simulink model "ConfiguredHevMmVirtualVehicle"  (R2025b)
settings: configuration reference "VehicleVariable" (kept outside this file)
StartFcn:
  | %tic
StopFcn:
  | %toc
model workspace (MAT data in the model file):
  ExtDrvCmdsSwitch : Simulink.Parameter (value not decoded)
  ExtDrvRefSwitch : Simulink.Parameter (value not decoded)
  ExtEnvSwitch : Simulink.Parameter (value not decoded)
  ExtGndSwitch : Simulink.Parameter (value not decoded)
symbols that are objects in the model workspace (value not decoded): ExtDrvCmdsSwitch, ExtDrvRefSwitch, ExtEnvSwitch, ExtGndSwitch
undefined symbols (not defined in the file or in its folder): AmbTemp, BaroPress, CurvGradRef, CurvRef, DCM, DriverAeroRes, DriverDrivelineRes, DriverInitialGear, DriverPreviewDist, DriverRollRes, DriverShiftTime, DriverTimeConst, DriverTractiveForce, EnvAbsPrs, EnvAirTemp, EnvGrvty, EnvNomFrictionScaling, EnvNominalGrade, EnvScnFrictionMap, EnvScnFrictionMapXBpts, EnvScnFrictionMapYBpts, EnvScnHeightMap, EnvScnHeightMapXBpts, EnvScnHeightMapYBpts, EnvWindVelX, EnvWindVelY, EnvWindVelZ, Gnd, Grade, HazzardCmd, HighBeamCmd, lambda_mux, LeftSignalCmd, LngRef, LowBeamCmd, LtrRef, PhiRef, PlntVehDstCGFrntAxl, PlntVehDstCGRearAxl, PlntVehInitLatPos, PlntVehInitLongPos, PlntVehInitPitchAng, PlntVehInitRollAng, PlntVehInitVertPos, PlntVehInitYawAng, PlntVehMass, PlntVehTrckWdth, PlntVehYawMomentInertia, PlntWhlLdRadiusFrnt, PlntWhlLdRadiusRear, RightSignalCmd, ScnCRRadius, Sim3dSensor, Wind, XRef, YRef, Z
libraries: simulink x28, autolibutils x8, autolibsharedcommon x7, vehdynlibscenariocommon x7, vehdynlibviscommon x4, vehdynlibdriver x2, sim3dgroundtruthsensorlib x2, sim3dlib x2, autolibshared x2, sim3dautolib x2, sl3dlib x1, sharedtransform x1
(part 2 of 6)

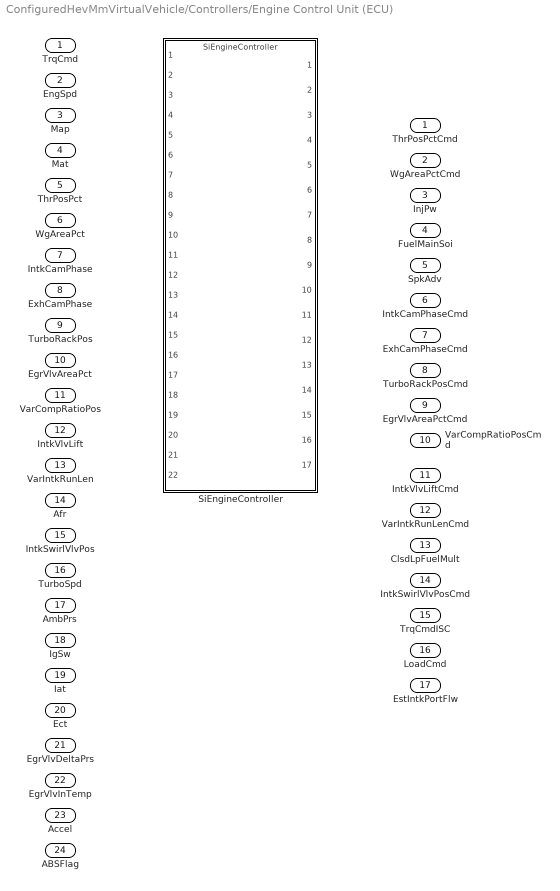
== system ConfiguredHevMmVirtualVehicle/Controllers/Engine Control Unit (ECU) ==
  TrqCmd : Inport
  EngSpd : Inport  Port=2
  Map : Inport  Port=3
  Mat : Inport  Port=4
  ThrPosPct : Inport  Port=5
  WgAreaPct : Inport  Port=6
  IntkCamPhase : Inport  Port=7
  ExhCamPhase : Inport  Port=8
  TurboRackPos : Inport  Port=9
  EgrVlvAreaPct : Inport  Port=10
  VarCompRatioPos : Inport  Port=11
  IntkVlvLift : Inport  Port=12
  VarIntkRunLen : Inport  Port=13
  Afr : Inport  Port=14
  IntkSwirlVlvPos : Inport  Port=15
  TurboSpd : Inport  Port=16  Unit=rpm
  AmbPrs : Inport  Port=17
  IgSw : Inport  Port=18
  Iat : Inport  Port=19
  Ect : Inport  Port=20
  EgrVlvDeltaPrs : Inport  Port=21
  EgrVlvInTemp : Inport  Port=22
  Accel : Inport  Port=23
  ABSFlag : Inport  Port=24
  SiEngineController : ModelReference  ModelNameDialog=SiEngineController  SimulationMode=Normal  VariantControl=SiEngineController  ModelReferenceVersion=11.0
  ThrPosPctCmd : Outport  VectorParamsAs1DForOutWhenUnconnected=off
  WgAreaPctCmd : Outport  Port=2  VectorParamsAs1DForOutWhenUnconnected=off
  InjPw : Outport  Port=3  VectorParamsAs1DForOutWhenUnconnected=off
  FuelMainSoi : Outport  Port=4  VectorParamsAs1DForOutWhenUnconnected=off
  SpkAdv : Outport  Port=5  VectorParamsAs1DForOutWhenUnconnected=off
  IntkCamPhaseCmd : Outport  Port=6  VectorParamsAs1DForOutWhenUnconnected=off
  ExhCamPhaseCmd : Outport  Port=7  VectorParamsAs1DForOutWhenUnconnected=off
  TurboRackPosCmd : Outport  Port=8  VectorParamsAs1DForOutWhenUnconnected=off
  EgrVlvAreaPctCmd : Outport  Port=9  VectorParamsAs1DForOutWhenUnconnected=off
  VarCompRatioPosCmd : Outport  Port=10  VectorParamsAs1DForOutWhenUnconnected=off
  IntkVlvLiftCmd : Outport  Port=11  VectorParamsAs1DForOutWhenUnconnected=off
  VarIntkRunLenCmd : Outport  Port=12  VectorParamsAs1DForOutWhenUnconnected=off
  ClsdLpFuelMult : Outport  Port=13  VectorParamsAs1DForOutWhenUnconnected=off
  IntkSwirlVlvPosCmd : Outport  Port=14  VectorParamsAs1DForOutWhenUnconnected=off
  TrqCmdISC : Outport  Port=15  VectorParamsAs1DForOutWhenUnconnected=off
  LoadCmd : Outport  Port=16  VectorParamsAs1DForOutWhenUnconnected=off
  EstIntkPortFlw : Outport  Port=17  VectorParamsAs1DForOutWhenUnconnected=off

== system ConfiguredHevMmVirtualVehicle/Controllers/TCU Input ==
  CntrlRx : Inport
  Brake : Inport  Port=2
  Bus Selector : BusSelector  OutputSignals=ABSFlag
  Bus Selector1 : BusSelector  OutputSignals=Driver.AccelFdbk,Driver.DecelFdbk,Driver.GearFdbk,Trans.Info.Eng.EngSpd,FrntWheels.Wheels.Omega,RearWheels.Wheels.Omega,Body.BdyFrm.Cg.Vel.xdot
  Bus to Vector : BusToVector
  Bus to Vector1 : BusToVector
  Ground : Ground
  Ground1 : Ground
  Rate Transition{1..8,23} (9 alike) : RateTransition  Deterministic=off
  Vector Concatenate : Concatenate
  <AccFdbk> : Outport
  <DecelFdbk> : Outport  Port=2
  <GearFdbk> : Outport  Port=3
  <EngSpd> : Outport  Port=4
  <Omega> : Outport  Port=5
  <Vehicle> : Outport  Port=6
  ABSFlag : Outport  Port=7
  UpReq : Outport  Port=8
  DnReq : Outport  Port=9
  wires:
  Bus Selector1/7 -> Rate Transition5/1  "<xdot>"
  Bus Selector1/2 -> Rate Transition1/1  "<DecelFdbk>"
  Ground/1 -> Rate Transition7/1
  CntrlRx/1 -> Bus Selector1/1
  Bus Selector1/1 -> Rate Transition23/1  "<AccelFdbk>"
  Vector Concatenate/1 -> Rate Transition4/1
  Bus Selector1/4 -> Rate Transition3/1  "<EngSpd>"
  Bus Selector1/3 -> Rate Transition2/1  "<GearFdbk>"
  Ground1/1 -> Rate Transition8/1
  Bus Selector/1 -> Rate Transition6/1  "<ABSFlag>"
  Brake/1 -> Bus Selector/1
  Rate Transition23/1 -> <AccFdbk>/1
  Rate Transition1/1 -> <DecelFdbk>/1
  Rate Transition2/1 -> <GearFdbk>/1
  Rate Transition3/1 -> <EngSpd>/1
  Rate Transition4/1 -> <Omega>/1
  Rate Transition5/1 -> <Vehicle>/1
  Rate Transition6/1 -> ABSFlag/1
  Rate Transition7/1 -> UpReq/1
  Rate Transition8/1 -> DnReq/1
  Bus Selector1/5 -> Bus to Vector/1  "<Omega>"
  Bus Selector1/6 -> Bus to Vector1/1  "<Omega>"
  Bus to Vector/1 -> Vector Concatenate/1
  Bus to Vector1/1 -> Vector Concatenate/2

== system ConfiguredHevMmVirtualVehicle/Controllers/TCU Output ==
  GearCmd : Inport
  Bus Creator1 : BusCreator  Inputs=1
  First Order Hold : FirstOrderHold  ErrorTolerance=inf
  Trans : Outport
  wires:
  Bus Creator1/1 -> Trans/1  "Trans"
  GearCmd/1 -> First Order Hold/1  "GearCmd"
  First Order Hold/1 -> Bus Creator1/1  "GearCmd"

== system ConfiguredHevMmVirtualVehicle/Controllers/Thermal Input ==
  Bus Element In : Inport  PortName=CntrlRx  Element=Thermal.BattCoolTemp
  Bus Element In2 : Inport  PortName=CntrlRx  Element=Thermal.CondPress
  Bus Element In5 : Inport  PortName=CntrlRx  Element=Thermal.MotorTemp
  Bus Element In6 : Inport  PortName=CntrlRx  Element=Thermal.BattTemp
  Bus Element In7 : Inport  PortName=CntrlRx  Element=Thermal.EMCoolTempOut
  BusElementIn2 : Inport  PortName=CntrlRx  Element=Thermal.ChlrPress
  Bus Element In1 : Inport  PortName=CntrlRx  Element=Battery.BMSSensors.CellTemperatures
  Bus Element In4 : Inport  PortName=CntrlRx  Element=Env.AmbTemp
  Rate Transition{,1,3..6,8,11} (8 alike) : RateTransition
  CoolTemp : Outport
  CellTemps : Outport  Port=2
  AmbTemp : Outport  Port=3
  CondPress : Outport  Port=4
  MotorTemp : Outport  Port=5
  BattTemp : Outport  Port=6
  EMCoolTempOut : Outport  Port=7
  ChlrPress : Outport  Port=8
  wires:
  Bus Element In/1 -> Rate Transition/1
  Bus Element In1/1 -> Rate Transition8/1
  Rate Transition/1 -> CoolTemp/1
  Bus Element In2/1 -> Rate Transition1/1
  Rate Transition1/1 -> CondPress/1
  Rate Transition3/1 -> AmbTemp/1
  Bus Element In4/1 -> Rate Transition3/1
  Rate Transition4/1 -> MotorTemp/1
  Bus Element In5/1 -> Rate Transition4/1
  Rate Transition5/1 -> BattTemp/1
  Bus Element In6/1 -> Rate Transition5/1
  Rate Transition6/1 -> EMCoolTempOut/1
  Bus Element In7/1 -> Rate Transition6/1
  Rate Transition8/1 -> CellTemps/1
  BusElementIn2/1 -> Rate Transition11/1
  Rate Transition11/1 -> ChlrPress/1

== system ConfiguredHevMmVirtualVehicle/Controllers/Thermal Management ==
  CoolTemp : Inport
  CellTemps : Inport  Port=2
  AmbTemp : Inport  Port=3  Unit=K
  CondPress : Inport  Port=4
  MotorTemp : Inport  Port=5
  BattTemp : Inport  Port=6
  EMCoolTempOut : Inport  Port=7
  ChlrPress : Inport  Port=8
  NoThermalControl : ModelReference  ModelNameDialog=NoThermalControl  SimulationMode=Normal  VariantControl=NoThermalControl  ModelReferenceVersion=5.0
  ValveCmd : Outport
  PumpCmd : Outport  Port=2
  CmpCmd : Outport  Port=3
  FanCmd : Outport  Port=4
  HeaterCmd : Outport  Port=5
  MotPmpCmd : Outport  Port=6
  BattPmpCmd : Outport  Port=7
  ChlrByPCmd : Outport  Port=8
  SerParCmd : Outport  Port=9
  RadByPCmd : Outport  Port=10

== system ConfiguredHevMmVirtualVehicle/Controllers/Thermal Output ==
  ValveCmd : Inport
  PumpCmd : Inport  Port=2
  CmpCmd : Inport  Port=3
  FanCmd : Inport  Port=4
  HeaterCmd : Inport  Port=5
  MotPmpCmd : Inport  Port=6
  BattPmpCmd : Inport  Port=7
  ChlrPyPCmd : Inport  Port=8
  SerParCmd : Inport  Port=9
  RadByPCmd : Inport  Port=10
  First Order Hold{,1..9} (10 alike) : FirstOrderHold  ErrorTolerance=inf
  Bus Element Out : Outport  PortName=Thermal  Element=ValveCmd
  Bus Element Out1 : Outport  PortName=Thermal  Element=PumpCmd
  Bus Element Out2 : Outport  PortName=Thermal  Element=CmpCmd
  Bus Element Out3 : Outport  PortName=Thermal  Element=FanCmd
  Bus Element Out4 : Outport  PortName=Thermal  Element=HeaterCmd
  Bus Element Out5 : Outport  PortName=Thermal  Element=MotPmpCmd
  Bus Element Out6 : Outport  PortName=Thermal  Element=BattPmpCmd
  Bus Element Out7 : Outport  PortName=Thermal  Element=ChlrByPCmd
  Bus Element Out8 : Outport  PortName=Thermal  Element=SerParCmd
  Bus Element Out9 : Outport  PortName=Thermal  Element=RadByPCmd
  wires:
  PumpCmd/1 -> First Order Hold1/1
  ValveCmd/1 -> First Order Hold/1
  First Order Hold/1 -> Bus Element Out/1
  First Order Hold1/1 -> Bus Element Out1/1
  CmpCmd/1 -> First Order Hold2/1
  First Order Hold2/1 -> Bus Element Out2/1
  First Order Hold3/1 -> Bus Element Out3/1
  FanCmd/1 -> First Order Hold3/1
  HeaterCmd/1 -> First Order Hold4/1
  First Order Hold4/1 -> Bus Element Out4/1
  MotPmpCmd/1 -> First Order Hold5/1
  First Order Hold5/1 -> Bus Element Out5/1
  BattPmpCmd/1 -> First Order Hold6/1
  First Order Hold6/1 -> Bus Element Out6/1
  ChlrPyPCmd/1 -> First Order Hold7/1
  First Order Hold7/1 -> Bus Element Out7/1
  First Order Hold8/1 -> Bus Element Out8/1
  SerParCmd/1 -> First Order Hold8/1
  First Order Hold9/1 -> Bus Element Out9/1
  RadByPCmd/1 -> First Order Hold9/1

== system ConfiguredHevMmVirtualVehicle/Controllers/Transmission Control Unit (TCU) ==
  Accel : Inport
  BrkCmd : Inport  Port=2
  GearReq : Inport  Port=3
  EngSpd : Inport  Port=4
  Omega : Inport  Port=5  Unit=rad/s
  VehSpdFdbk : Inport  Port=6
  ABSFlag : Inport  Port=7
  UpReq : Inport  Port=8
  DownReq : Inport  Port=9  Unit=rad/s
  DriverPassThrough : ModelReference  ModelNameDialog=DriverPassThrough  SimulationMode=Normal  VariantControl=DriverPassThrough  ModelReferenceVersion=11.0
  " Gear" : Outport  VectorParamsAs1DForOutWhenUnconnected=off

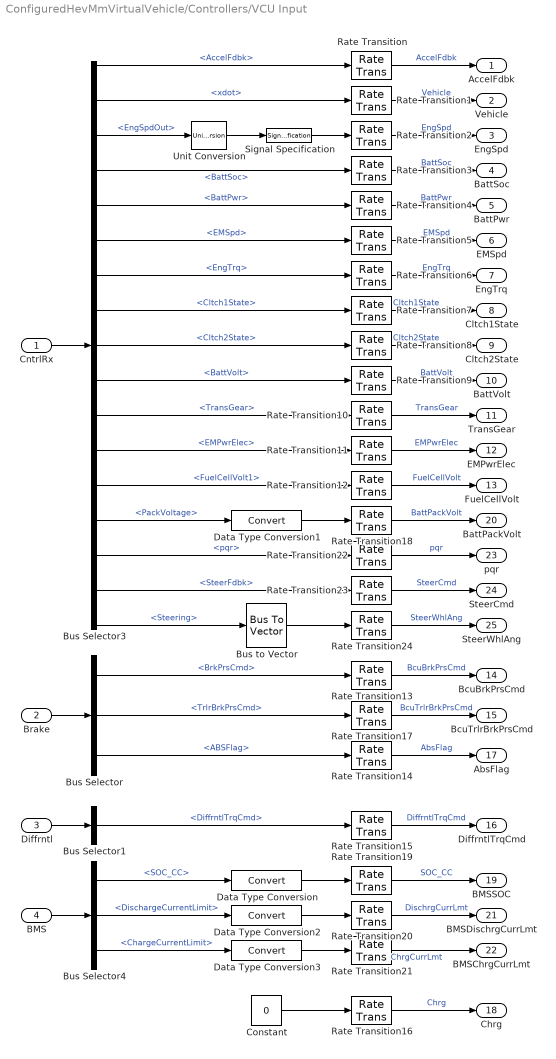
== system ConfiguredHevMmVirtualVehicle/Controllers/VCU Input ==
  CntrlRx : Inport
  Brake : Inport  Port=2
  Diffrntl : Inport  Port=3
  BMS : Inport  Port=4
  Bus Selector : BusSelector  OutputSignals=BrkPrsCmd,TrlrBrkPrsCmd,ABSFlag
  Bus Selector1 : BusSelector  OutputSignals=DiffrntlTrqCmd
  Bus Selector3 : BusSelector  OutputSignals=Driver.AccelFdbk,Body.BdyFrm.Cg.Vel.xdot,Engine.EngSpdOut,Battery.BattInfo.BattSoc,Battery.BattInfo.BattPwr,EM.EMSpd,Engine.EngTrq,Trans.Cltch1State,Trans.Cltch2State,Battery.BattInfo.BattVolt,Trans.Info.Trans.TransGear,EM.EMPwrElec,FuelCell.FuelCellVolt1,Battery.BMSSensors.PackVoltage,IMU.pqr,Driver.SteerFdbk,Steering
  Bus Selector4 : BusSelector  OutputSignals=BMSInfo.SOC.SOC_CC,BMSCmd.CurrentLimitsBus.DischargeCurrentLimit,BMSCmd.CurrentLimitsBus.ChargeCurrentLimit
  Bus to Vector : BusToVector
  Constant : Constant  Value=0  SampleTime=-1
  Data Type Conversion{,1..3} (4 alike) : DataTypeConversion  SaturateOnIntegerOverflow=off  RndMeth=Floor
  Rate Transition{,1..24} (25 alike) : RateTransition  Deterministic=off
  Signal Specification : SignalSpecification  Unit=rad/s
  Unit Conversion : UnitConversion
  AccelFdbk : Outport
  Vehicle : Outport  Port=2
  EngSpd : Outport  Port=3
  BattSoc : Outport  Port=4
  BattPwr : Outport  Port=5
  EMSpd : Outport  Port=6
  EngTrq : Outport  Port=7
  Cltch1State : Outport  Port=8
  Cltch2State : Outport  Port=9
  BattVolt : Outport  Port=10
  TransGear : Outport  Port=11
  EMPwrElec : Outport  Port=12
  FuelCellVolt : Outport  Port=13
  BcuBrkPrsCmd : Outport  Port=14
  BcuTrlrBrkPrsCmd : Outport  Port=15
  DiffrntlTrqCmd : Outport  Port=16
  AbsFlag : Outport  Port=17
  Chrg : Outport  Port=18
  BMSSOC : Outport  Port=19
  BattPackVolt : Outport  Port=20
  BMSDischrgCurrLmt : Outport  Port=21
  BMSChrgCurrLmt : Outport  Port=22
  pqr : Outport  Port=23
  SteerCmd : Outport  Port=24
  SteerWhlAng : Outport  Port=25
  wires:
  Bus Selector3/5 -> Rate Transition4/1  "<BattPwr>"
  Bus Selector3/1 -> Rate Transition/1  "<AccelFdbk>"
  Bus Selector3/7 -> Rate Transition6/1  "<EngTrq>"
  Bus Selector3/4 -> Rate Transition3/1  "<BattSoc>"
  Bus Selector3/6 -> Rate Transition5/1  "<EMSpd>"
  CntrlRx/1 -> Bus Selector3/1
  Bus Selector3/11 -> Rate Transition10/1  "<TransGear>"
  Bus Selector3/9 -> Rate Transition8/1  "<Cltch2State>"
  Bus Selector3/13 -> Rate Transition12/1  "<FuelCellVolt1>"
  Bus Selector3/2 -> Rate Transition1/1  "<xdot>"
  Bus Selector3/8 -> Rate Transition7/1  "<Cltch1State>"
  Bus Selector3/10 -> Rate Transition9/1  "<BattVolt>"
  Bus Selector3/3 -> Unit Conversion/1  "<EngSpdOut>"
  Bus Selector3/12 -> Rate Transition11/1  "<EMPwrElec>"
  Bus Selector/1 -> Rate Transition13/1  "<BrkPrsCmd>"
  Constant/1 -> Rate Transition16/1
  Brake/1 -> Bus Selector/1
  Bus Selector/3 -> Rate Transition14/1  "<ABSFlag>"
  Diffrntl/1 -> Bus Selector1/1
  Bus Selector1/1 -> Rate Transition15/1  "<DiffrntlTrqCmd>"
  Rate Transition/1 -> AccelFdbk/1  "AccelFdbk"
  Rate Transition1/1 -> Vehicle/1  "Vehicle"
  Rate Transition2/1 -> EngSpd/1  "EngSpd"
  Rate Transition3/1 -> BattSoc/1  "BattSoc"
  Rate Transition4/1 -> BattPwr/1  "BattPwr"
  Rate Transition5/1 -> EMSpd/1  "EMSpd"
  Rate Transition6/1 -> EngTrq/1  "EngTrq"
  Rate Transition7/1 -> Cltch1State/1  "Cltch1State"
  Rate Transition8/1 -> Cltch2State/1  "Cltch2State"
  Rate Transition9/1 -> BattVolt/1  "BattVolt"
  Rate Transition10/1 -> TransGear/1  "TransGear"
  Rate Transition11/1 -> EMPwrElec/1  "EMPwrElec"
  Rate Transition12/1 -> FuelCellVolt/1  "FuelCellVolt"
  Rate Transition13/1 -> BcuBrkPrsCmd/1  "BcuBrkPrsCmd"
  Rate Transition14/1 -> AbsFlag/1  "AbsFlag"
  Rate Transition15/1 -> DiffrntlTrqCmd/1  "DiffrntlTrqCmd"
  Rate Transition16/1 -> Chrg/1  "Chrg"
  Rate Transition20/1 -> BMSDischrgCurrLmt/1  "DischrgCurrLmt"
  Rate Transition19/1 -> BMSSOC/1  "SOC_CC"
  Rate Transition21/1 -> BMSChrgCurrLmt/1  "ChrgCurrLmt"
  Data Type Conversion3/1 -> Rate Transition21/1
  Data Type Conversion2/1 -> Rate Transition20/1
  Bus Selector4/1 -> Data Type Conversion/1  "<SOC_CC>"
  Data Type Conversion/1 -> Rate Transition19/1
  Bus Selector4/3 -> Data Type Conversion3/1  "<ChargeCurrentLimit>"
  Bus Selector4/2 -> Data Type Conversion2/1  "<DischargeCurrentLimit>"
  BMS/1 -> Bus Selector4/1
  Data Type Conversion1/1 -> Rate Transition18/1
  Rate Transition18/1 -> BattPackVolt/1  "BattPackVolt"
  Bus Selector3/14 -> Data Type Conversion1/1  "<PackVoltage>"
  Bus Selector/2 -> Rate Transition17/1  "<TrlrBrkPrsCmd>"
  Rate Transition17/1 -> BcuTrlrBrkPrsCmd/1  "BcuTrlrBrkPrsCmd"
  Rate Transition22/1 -> pqr/1  "pqr"
  Rate Transition23/1 -> SteerCmd/1  "SteerCmd"
  Rate Transition24/1 -> SteerWhlAng/1  "SteerWhlAng"
  Bus Selector3/15 -> Rate Transition22/1  "<pqr>"
  Bus Selector3/16 -> Rate Transition23/1  "<SteerFdbk>"
  Bus Selector3/17 -> Bus to Vector/1  "<Steering>"
  Unit Conversion/1 -> Signal Specification/1
  Signal Specification/1 -> Rate Transition2/1
  Bus to Vector/1 -> Rate Transition24/1

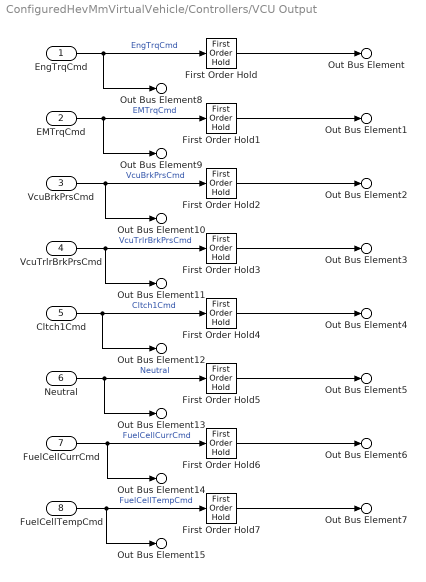
== system ConfiguredHevMmVirtualVehicle/Controllers/VCU Output ==
  EngTrqCmd : Inport
  EMTrqCmd : Inport  Port=2
  VcuBrkPrsCmd : Inport  Port=3
  VcuTrlrBrkPrsCmd : Inport  Port=4
  Cltch1Cmd : Inport  Port=5
  Neutral : Inport  Port=6
  FuelCellCurrCmd : Inport  Port=7
  FuelCellTempCmd : Inport  Port=8
  First Order Hold{,1..2,4..7} (7 alike) : FirstOrderHold  ErrorTolerance=inf
  First Order Hold3 : FirstOrderHold  ErrorTolerance=inf  AllowContinuousInput=on
  Out Bus Element : Outport  PortName=Vcu  Element=EngTrqCmd
  Out Bus Element1 : Outport  PortName=Vcu  Element=EMTrqCmd
  Out Bus Element2 : Outport  PortName=Vcu  Element=VcuBrkPrsCmd
  Out Bus Element3 : Outport  PortName=Vcu  Element=VcuTrlrBrkPrsCmd
  Out Bus Element4 : Outport  PortName=Vcu  Element=Cltch1Cmd
  Out Bus Element5 : Outport  PortName=Vcu  Element=Neutral
  Out Bus Element6 : Outport  PortName=Vcu  Element=FuelCellCurrCmd
  Out Bus Element7 : Outport  PortName=Vcu  Element=FuelCellTempCmd
  Out Bus Element8 : Outport  Port=2  PortName=VcuFdbk  Element=EngTrqCmd
  Out Bus Element9 : Outport  Port=2  PortName=VcuFdbk  Element=EMTrqCmd
  Out Bus Element10 : Outport  Port=2  PortName=VcuFdbk  Element=VcuBrkPrsCmd
  Out Bus Element11 : Outport  Port=2  PortName=VcuFdbk  Element=VcuTrlrBrkPrsCmd
  Out Bus Element12 : Outport  Port=2  PortName=VcuFdbk  Element=Cltch1Cmd
  Out Bus Element13 : Outport  Port=2  PortName=VcuFdbk  Element=Neutral
  Out Bus Element14 : Outport  Port=2  PortName=VcuFdbk  Element=FuelCellCurrCmd
  Out Bus Element15 : Outport  Port=2  PortName=VcuFdbk  Element=FuelCellTempCmd
  wires:
  Cltch1Cmd/1 -> Out Bus Element12/1, First Order Hold4/1  "Cltch1Cmd"
  EngTrqCmd/1 -> Out Bus Element8/1, First Order Hold/1  "EngTrqCmd"
  VcuBrkPrsCmd/1 -> Out Bus Element10/1, First Order Hold2/1  "VcuBrkPrsCmd"
  Neutral/1 -> Out Bus Element13/1, First Order Hold5/1  "Neutral"
  FuelCellCurrCmd/1 -> Out Bus Element14/1, First Order Hold6/1  "FuelCellCurrCmd"
  EMTrqCmd/1 -> Out Bus Element9/1, First Order Hold1/1  "EMTrqCmd"
  FuelCellTempCmd/1 -> Out Bus Element15/1, First Order Hold7/1  "FuelCellTempCmd"
  VcuTrlrBrkPrsCmd/1 -> Out Bus Element11/1, First Order Hold3/1  "VcuTrlrBrkPrsCmd"
  First Order Hold/1 -> Out Bus Element/1
  First Order Hold1/1 -> Out Bus Element1/1
  First Order Hold2/1 -> Out Bus Element2/1
  First Order Hold3/1 -> Out Bus Element3/1
  First Order Hold4/1 -> Out Bus Element4/1
  First Order Hold5/1 -> Out Bus Element5/1
  First Order Hold6/1 -> Out Bus Element6/1
  First Order Hold7/1 -> Out Bus Element7/1

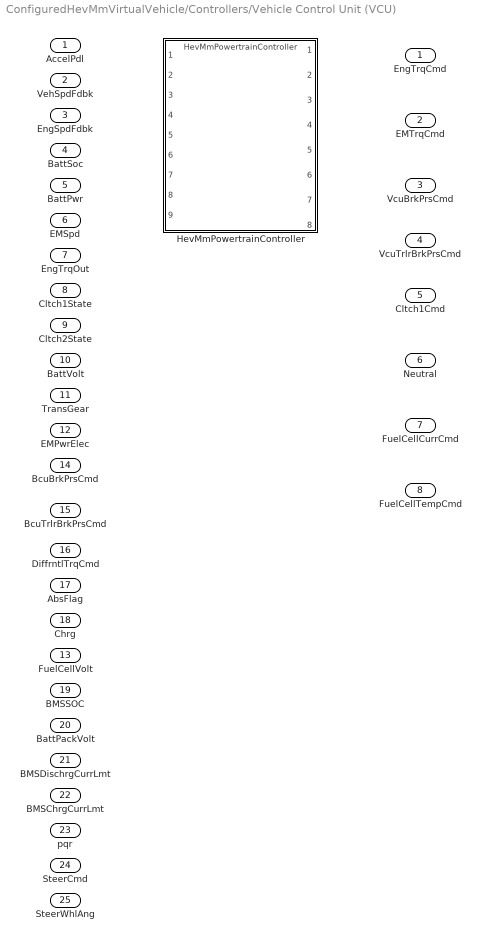
== system ConfiguredHevMmVirtualVehicle/Controllers/Vehicle Control Unit (VCU) ==
  AccelPdl : Inport
  VehSpdFdbk : Inport  Port=2
  EngSpdFdbk : Inport  Port=3
  BattSoc : Inport  Port=4
  BattPwr : Inport  Port=5
  EMSpd : Inport  Port=6
  EngTrqOut : Inport  Port=7
  Cltch1State : Inport  Port=8
  Cltch2State : Inport  Port=9
  BattVolt : Inport  Port=10
  TransGear : Inport  Port=11
  EMPwrElec : Inport  Port=12
  FuelCellVolt : Inport  Port=13
  BcuBrkPrsCmd : Inport  Port=14
  BcuTrlrBrkPrsCmd : Inport  Port=15
  DiffrntlTrqCmd : Inport  Port=16
  AbsFlag : Inport  Port=17
  Chrg : Inport  Port=18
  BMSSOC : Inport  Port=19
  BattPackVolt : Inport  Port=20
  BMSDischrgCurrLmt : Inport  Port=21
  BMSChrgCurrLmt : Inport  Port=22
  pqr : Inport  Port=23
  SteerCmd : Inport  Port=24
  SteerWhlAng : Inport  Port=25
  HevMmPowertrainController : ModelReference  ModelNameDialog=HevMmPowertrainController  SimulationMode=Normal  VariantControl=HevMmPowertrainController  ModelReferenceVersion=16.0
  EngTrqCmd : Outport  VectorParamsAs1DForOutWhenUnconnected=off
  EMTrqCmd : Outport  Port=2  VectorParamsAs1DForOutWhenUnconnected=off
  VcuBrkPrsCmd : Outport  Port=3  VectorParamsAs1DForOutWhenUnconnected=off
  VcuTrlrBrkPrsCmd : Outport  Port=4  VectorParamsAs1DForOutWhenUnconnected=off
  Cltch1Cmd : Outport  Port=5  VectorParamsAs1DForOutWhenUnconnected=off
  Neutral : Outport  Port=6  VectorParamsAs1DForOutWhenUnconnected=off
  FuelCellCurrCmd : Outport  Port=7  VectorParamsAs1DForOutWhenUnconnected=off
  FuelCellTempCmd : Outport  Port=8  VectorParamsAs1DForOutWhenUnconnected=off

== system ConfiguredHevMmVirtualVehicle/Driver Commands/Driver Commands ==
  VehRef : Inport
  VehFdbk : Inport  Port=2
  Env : Inport  Port=3
  SteerCmd : Inport  Port=4
  AccelCmd : Inport  Port=5
  BrakeCmd : Inport  Port=6
  GearCmd : Inport  Port=7
  Dashboard Widgets : Subsystem  VariantControl=Dashboard Widgets
  Game Wheel Hardware : Subsystem  VariantControl=Game Wheel Hardware
  Longitudinal Driver : Subsystem  VariantControl=Longitudinal Driver
  No Driver : Subsystem  VariantControl=No Driver
  Open Loop : Subsystem  VariantControl=Open Loop
  Predictive Driver : Subsystem  VariantControl=Predictive Driver
  Predictive Stanley Driver : Subsystem  VariantControl=Predictive Stanley Driver
  " Driver" : Outport  VectorParamsAs1DForOutWhenUnconnected=off

== system ConfiguredHevMmVirtualVehicle/Environment/Ground Feedback ==
  WheelFdbk : Inport
  InertFrm : Inport  Port=2
  3D Engine : Subsystem  VariantControl=1
  Constant : Subsystem  VariantControl=0
  Height Map : Subsystem  VariantControl=3
  Ideal Inclined Plane : Subsystem  VariantControl=4
  Three-Axle Constant : Subsystem  VariantControl=2
  Z : Outport  VectorParamsAs1DForOutWhenUnconnected=off
  DCM : Outport  Port=2  VectorParamsAs1DForOutWhenUnconnected=off

== system ConfiguredHevMmVirtualVehicle/Environment/Subsystem ==
  ExtEnv : Inport
  ExtGnd : Inport  Port=2
  AmbTemp : Inport  Port=3
  BaroPress : Inport  Port=4
  Wind : Inport  Port=5
  InGnd : Inport  Port=6
  Bus Assignment : BusAssignment  AssignedSignals=AmbTemp,BaroPress,Wind,Grade
  Bus Assignment1 : BusAssignment  AssignedSignals=Z,DCM,lambda_mux
  Bus Assignment2 : BusAssignment  AssignedSignals=BaroPress,AmbTemp,Wind,Grade,Gnd
  Bus Selector : BusSelector  OutputSignals=BaroPress,AmbTemp,Wind,Grade
  Estimated Grade : Subsystem
  ExtEnvSwitch : Constant  Value=ExtEnvSwitch  SampleTime=-1
  ExtGndSwitch : Constant  Value=ExtGndSwitch  SampleTime=-1
  Switch : Switch  Criteria=u2 > Threshold  SaturateOnIntegerOverflow=off  InputSameDT=off
  Switch1 : Switch  Criteria=u2 > Threshold  SaturateOnIntegerOverflow=off  InputSameDT=off
  To Virtual Bus : SignalConversion  ConversionOutput=Virtual bus  OverrideOpt=off
  VVCEnv : Constant  Value=0  OutDataTypeStr=Bus: VVCEnvGndBUS  SampleTime=-1
  Variant Subsystem : Subsystem  Variant=on  VariantControlMode=label  LabelModeActiveChoice=TwoAxle
  Env : Outport
  wires:
  Bus Assignment1/1 -> Switch1/3
  Estimated Grade/1(Grade) -> Bus Assignment/5
  ExtGndSwitch/1 -> Switch1/2
  ExtEnv/1 -> Switch/1, Bus Assignment/1
  InGnd/1 -> Variant Subsystem/1(InGnd), Estimated Grade/1(Gnd)
  ExtEnvSwitch/1 -> Switch/2
  Bus Assignment/1 -> Switch/3
  BaroPress/1 -> Bus Assignment/3
  VVCEnv/1 -> Bus Assignment2/1
  Switch1/1 -> Bus Assignment2/6
  ExtGnd/1 -> Switch1/1, Bus Assignment1/1
  Wind/1 -> Bus Assignment/4
  Bus Selector/1 -> Bus Assignment2/2  "<BaroPress>"
  Switch/1 -> Bus Selector/1
  Bus Selector/2 -> Bus Assignment2/3  "<AmbTemp>"
  Bus Assignment2/1 -> To Virtual Bus/1
  Bus Selector/4 -> Bus Assignment2/5  "<Grade>"
  Bus Selector/3 -> Bus Assignment2/4  "<Wind>"
  AmbTemp/1 -> Bus Assignment/2
  To Virtual Bus/1 -> Env/1
  Variant Subsystem/1(z) -> Bus Assignment1/2
  Variant Subsystem/2(<DCM>) -> Bus Assignment1/3
  Variant Subsystem/3(lambda_mux) -> Bus Assignment1/4

== system ConfiguredHevMmVirtualVehicle/Environment/Varying Friction ==
  InertFrm : Inport
  Cg : Inport  Port=2
  Constant Friction : Subsystem  VariantControl=0
  Friction Map : Subsystem  VariantControl=3
  Three-Axle Constant Friction : Subsystem  VariantControl=2
  Varying Friction : Subsystem  VariantControl=1
  FricCoeffLambda : Outport

== system ConfiguredHevMmVirtualVehicle/Scenarios/Coordinate Systems ==
  ExtDrvRefIn : Inport
  ExtDrvCmdIn : Inport  Port=2
  ISO 8855 (Z-up) : Subsystem  VariantControl=Choice
  SAE J670 (Z-down) : Subsystem  VariantControl=ISO 8855 (Z-up)1
  ExtDrvRef : Outport
  ExtDrvCmd : Outport  Port=2

== system ConfiguredHevMmVirtualVehicle/Scenarios/Reference Generator ==
  note: 1) Add Subsystem or Model blocks as valid variant choices.
      | 2) You cannot connect blocks at this level. At simulation, connectivity is automatically
      | determined, based on the active variant and port name matching.
  "VehFdbk " : Inport
  Braking : Subsystem  VariantControl=Braking
  Constant Radius : Subsystem  VariantControl=Constant Radius
  Double Lane Change : Subsystem  VariantControl=Double Lane Change
  Drive Cycle : Subsystem  VariantControl=Drive Cycle
  Fishhook : Subsystem  VariantControl=Fishhook
  Increasing Steer : Subsystem  VariantControl=Increasing Steer
  No Commands : Subsystem  VariantControl=No Commands
  Sine with Dwell : Subsystem  VariantControl=Sine with Dwell
  Swept Sine : Subsystem  VariantControl=Swept Sine
  WOT : Subsystem  VariantControl=Wide Open Throttle
  DrvRef : Outport  VectorParamsAs1DForOutWhenUnconnected=off
  DrvCmd : Outport  Port=2  VectorParamsAs1DForOutWhenUnconnected=off
  " Vis" : Outport  Port=3  VectorParamsAs1DForOutWhenUnconnected=off
  " Fdbk" : Outport  Port=4  VectorParamsAs1DForOutWhenUnconnected=off

== system ConfiguredHevMmVirtualVehicle/Scenarios/Reference Routing ==
  ExtDrvRef : Inport  OutDataTypeStr=Bus: VVCDrvRefBUS
  ExtDrvCmds : Inport  Port=2  OutDataTypeStr=Bus: VVCDrvCmdBUS
  DrvRef : Inport  Port=3
  DrvCmd : Inport  Port=4
  Bus Assignment : BusAssignment  AssignedSignals=LngRef,LtrRef,XRef,YRef,PhiRef,CurvRef
  Bus Assignment1 : BusAssignment  AssignedSignals=SteerCmd.EnblSteerCmd,SteerCmd.SteerCmd,SteerCmd.SteerHld,SteerCmd.SteerZero,AccelCmd.EnblAccelCmd,AccelCmd.AccelCmd,AccelCmd.AccelHld,AccelCmd.AccelZero,DecelCmd.EnblDecelCmd,DecelCmd.DecelCmd,DecelCmd.DecelHld,DecelCmd.DecelZero,TransCmd.TransModeCmd,TransCmd.GearCmd,TransCmd.UpShiftCmd,TransCmd.DwnShiftCmd,TransCmd.ClutchCmd
  Bus Creator : BusCreator  Inputs=2
  Bus Selector : BusSelector  OutputSignals=LngRef,LtrRef,XRef,YRef,PhiRef,CurvRef
  Bus Selector1 : BusSelector  OutputSignals=SteerCmd.EnblSteerCmd,SteerCmd.SteerCmd,SteerCmd.SteerHld,SteerCmd.SteerZero,AccelCmd.EnableAccelCmd,AccelCmd.AccelCmd,AccelCmd.AccelHld,AccelCmd.AccelZero,DecelCmd.EnblDecelCmd,DecelCmd.DecelCmd,DecelCmd.DecelHld,DecelCmd.DecelZero,TransCmd.TransModeCmd,TransCmd.GearCmd,TransCmd.UpShiftCmd,TransCmd.DwnShiftCmd,TransCmd.ClutchCmd
  ExtDrvCmdsSwitch : Constant  Value=ExtDrvCmdsSwitch
  ExtDrvRefSwitch : Constant  Value=ExtDrvRefSwitch
  Switch : Switch  Criteria=u2 > Threshold  SaturateOnIntegerOverflow=off  InputSameDT=off
  Switch1 : Switch  Criteria=u2 > Threshold  SaturateOnIntegerOverflow=off  InputSameDT=off
  Unit Conversion1 : UnitConversion
  VehRef : Outport
  wires:
  Bus Selector1/9 -> Bus Assignment1/10  "<EnblDecelCmd>"
  Bus Selector/1 -> Bus Assignment/2  "<LngRef>"
  Bus Selector1/8 -> Bus Assignment1/9  "<AccelZero>"
  Bus Selector1/4 -> Bus Assignment1/5  "<SteerZero>"
  Bus Selector1/3 -> Bus Assignment1/4  "<SteerHld>"
  Bus Selector1/10 -> Bus Assignment1/11  "<DecelCmd>"
  ExtDrvRef/1 -> Bus Assignment/1, Switch/1
  Bus Selector1/1 -> Bus Assignment1/2  "<EnblSteerCmd>"
  Bus Assignment/1 -> Switch/3
  Bus Assignment1/1 -> Switch1/3
  Bus Selector/2 -> Bus Assignment/3  "<LtrRef>"
  Bus Selector1/7 -> Bus Assignment1/8  "<AccelHld>"
  DrvRef/1 -> Bus Selector/1
  Switch1/1 -> Bus Creator/2  "DrvCmd"
  Bus Selector1/12 -> Bus Assignment1/13  "<DecelZero>"
  Bus Selector1/11 -> Bus Assignment1/12  "<DecelHld>"
  Bus Selector1/2 -> Unit Conversion1/1  "<SteerCmd>"
  Bus Selector1/6 -> Bus Assignment1/7  "<AccelCmd>"
  ExtDrvCmds/1 -> Bus Assignment1/1, Switch1/1
  ExtDrvRefSwitch/1 -> Switch/2
  ExtDrvCmdsSwitch/1 -> Switch1/2
  Switch/1 -> Bus Creator/1  "DrvRef"
  Bus Selector/6 -> Bus Assignment/7  "<CurvRef>"
  Bus Selector1/5 -> Bus Assignment1/6  "<EnableAccelCmd>"
  Bus Creator/1 -> VehRef/1  "VehRef"
  Unit Conversion1/1 -> Bus Assignment1/3
  DrvCmd/1 -> Bus Selector1/1
  Bus Selector/3 -> Bus Assignment/4  "<XRef>"
  Bus Selector/4 -> Bus Assignment/5  "<YRef>"
  Bus Selector/5 -> Bus Assignment/6  "<PhiRef>"
  Bus Selector1/13 -> Bus Assignment1/14  "<TransModeCmd>"
  Bus Selector1/14 -> Bus Assignment1/15  "<GearCmd>"
  Bus Selector1/15 -> Bus Assignment1/16  "<UpShiftCmd>"
  Bus Selector1/16 -> Bus Assignment1/17  "<DwnShiftCmd>"
  Bus Selector1/17 -> Bus Assignment1/18  "<ClutchCmd>"

== system ConfiguredHevMmVirtualVehicle/Visualization/3D Engine ==
  note: 1) Add Subsystem or Model blocks as valid variant choices.
      | 2) You cannot connect blocks at this level. At simulation, connectivity is automatically
      | determined, based on the active variant and port name matching.
  VehFdbk : Inport
  3D Engine : Subsystem  VariantControl=Engine3D
  3D Engine Disabled : Subsystem  VariantControl=NoEngine3D

== system ConfiguredHevMmVirtualVehicle/Visualization/Coordinate Systems ==
  VehFdbkIn : Inport
  ISO 8855 (Z-up) : Subsystem  VariantControl=Choice
  SAE J670 (Z-down) : Subsystem  VariantControl=ISO 8855 (Z-up)1
  VehFdbk : Outport

== system ConfiguredHevMmVirtualVehicle/Visualization/DataLogging ==
  VehFdbk : Inport
  Bus Selector : BusSelector  OutputSignals=Battery.BattInfo.BattSoc,Battery.BattInfo.BattVolt,Battery.BattInfo.BattCurr,Body.BdyFrm.Cg.Vel.xdot,Body.BdyFrm.Cg.Acc.ax,Body.BdyFrm.Cg.Acc.ay,Body.BdyFrm.Cg.Acc.az,Driver.SteerFdbk,Driver.AccelFdbk,Driver.DecelFdbk,Driver.GearFdbk,EM.EMSpd,EM.EMTrq,Engine.EngTrq,Engine.EngSpdOut
  Terminator{,1..14} (15 alike) : Terminator
  wires:
  Bus Selector/2 -> Terminator1/1  "<BattVolt>"
  VehFdbk/1 -> Bus Selector/1
  Bus Selector/1 -> Terminator/1  "<BattSoc>"
  Bus Selector/4 -> Terminator3/1  "<xdot>"
  Bus Selector/6 -> Terminator5/1  "<ay>"
  Bus Selector/9 -> Terminator8/1  "<AccelFdbk>"
  Bus Selector/5 -> Terminator4/1  "<ax>"
  Bus Selector/3 -> Terminator2/1  "<BattCurr>"
  Bus Selector/15 -> Terminator14/1  "<EngSpdOut>"
  Bus Selector/11 -> Terminator10/1  "<GearFdbk>"
  Bus Selector/7 -> Terminator6/1  "<az>"
  Bus Selector/12 -> Terminator11/1  "<EMSpd>"
  Bus Selector/8 -> Terminator7/1  "<SteerFdbk>"
  Bus Selector/14 -> Terminator13/1  "<EngTrq>"
  Bus Selector/10 -> Terminator9/1  "<DecelFdbk>"
  Bus Selector/13 -> Terminator12/1  "<EMTrq>"

== system ConfiguredHevMmVirtualVehicle/Visualization/Emission Calculations ==
  VehSpd : Inport
  TP HC Mass Flow : Inport  Port=2
  TP CO Mass Flow : Inport  Port=3
  TP NOx Mass Flow : Inport  Port=4
  TP CO2 Mass Flow : Inport  Port=5
  Integrator{,1..4} (5 alike) : Integrator
  Kg to g : Gain  Gain=1000
  "Kg to g " : Gain  Gain=1000
  "Kg to g  " : Gain  Gain=1000
  "Kg to g   " : Gain  Gain=1000
  L/100 Km Calc{,1..3} (4 alike) : Product  Inputs=/*
  Rate Transition{,1..3} (4 alike) : RateTransition  Deterministic=off
  Saturation : Saturate  UpperLimit=Inf  LowerLimit=0.2  ZeroCross=off
  Saturation1 : Saturate  UpperLimit=Inf  LowerLimit=1  ZeroCross=off
  Signal Specification5 : SignalSpecification  Unit=m/s
  Unit Conversion5 : UnitConversion
  m to km : Gain  Gain=0.001
  m to mi : Gain  Gain=0.000621371
  TP HC Mass : Outport  VectorParamsAs1DForOutWhenUnconnected=off
  TP CO Mass : Outport  Port=2  VectorParamsAs1DForOutWhenUnconnected=off
  TP NOx Mass : Outport  Port=3  VectorParamsAs1DForOutWhenUnconnected=off
  TP CO2 Mass : Outport  Port=4  VectorParamsAs1DForOutWhenUnconnected=off
  wires:
  L/100 Km Calc/1 -> Rate Transition/1
  m to mi/1 -> Saturation/1
  Saturation/1 -> L/100 Km Calc2/1, L/100 Km Calc1/1, L/100 Km Calc/1
  TP HC Mass Flow/1 -> Integrator1/1
  Integrator1/1 -> Kg to g/1
  Integrator/1 -> m to km/1, m to mi/1
  Kg to g/1 -> L/100 Km Calc/2
  TP CO Mass Flow/1 -> Integrator2/1
  Integrator2/1 -> "Kg to g "/1
  "Kg to g "/1 -> L/100 Km Calc1/2
  TP NOx Mass Flow/1 -> Integrator3/1
  Integrator3/1 -> "Kg to g  "/1
  "Kg to g  "/1 -> L/100 Km Calc2/2
  L/100 Km Calc1/1 -> Rate Transition1/1
  L/100 Km Calc2/1 -> Rate Transition2/1
  TP CO2 Mass Flow/1 -> Integrator4/1
  Integrator4/1 -> "Kg to g   "/1
  "Kg to g   "/1 -> L/100 Km Calc3/2
  L/100 Km Calc3/1 -> Rate Transition3/1
  Saturation1/1 -> L/100 Km Calc3/1
  m to km/1 -> Saturation1/1
  Rate Transition/1 -> TP HC Mass/1  "TP HC Mass (g/mi)"
  Rate Transition1/1 -> TP CO Mass/1  "TP CO Mass (g/mi)"
  Rate Transition2/1 -> TP NOx Mass/1  "TP NOx Mass (g/mi)"
  Rate Transition3/1 -> TP CO2 Mass/1  "TP CO2 Mass (g/km)"
  Unit Conversion5/1 -> Signal Specification5/1
  VehSpd/1 -> Unit Conversion5/1
  Signal Specification5/1 -> Integrator/1

== system ConfiguredHevMmVirtualVehicle/Visualization/External Output Routing ==
  VehFdbk : Inport
  Bus Assignment : BusAssignment  AssignedSignals=Driver.SteerFdbk,Driver.AccelFdbk,Driver.DecelFdbk,Driver.GearFdbk,Driver.IgnFdbk,Driveline.EngSpd,Driveline.TransGear,Body.InertFrm.Cg.Disp.X,Body.InertFrm.Cg.Disp.Y,Body.InertFrm.Cg.Disp.Z,Body.InertFrm.Cg.Vel.Xdot,Body.InertFrm.Cg.Vel.Ydot,Body.InertFrm.Cg.Vel.Zdot,Body.InertFrm.Cg.Ang.phi,Body.InertFrm.Cg.Ang.theta,Body.InertFrm.Cg.Ang.psi,Body.InertFrm.Geom.Disp.X,Body.InertFrm.Geom.Disp.Y,Body.InertFrm.Geom.Disp.Z,Body.InertFrm.Geom.Vel.Xdot,Body.InertFrm.Geom.Vel.Ydot,Body.InertFrm.Geom.Vel.Zdot,Body.BdyFrm.Cg.Vel.xdot,Body.BdyFrm.Cg.Vel.ydot,Body.BdyFrm.Cg.Vel.zdot,Body.BdyFrm.Cg.AngVel.p,Body.BdyFrm.Cg.AngVel.q,Body.BdyFrm.Cg.AngVel.r,Body.BdyFrm.Cg.Acc.ax,Body.BdyFrm.Cg.Acc.ay,Body.BdyFrm.Cg.Acc.az,Body.BdyFrm.Cg.Acc.xddot,Body.BdyFrm.Cg.Acc.yddot,Body.BdyFrm.Cg.Acc.zddot,Body.BdyFrm.Cg.AngAcc.pdot,Body.BdyFrm.Cg.AngAcc.qdot,Body.BdyFrm.Cg.AngAcc.rdot
  Bus Selector1 : BusSelector  OutputSignals=Driver.SteerFdbk,Driver.AccelFdbk,Driver.DecelFdbk,Driver.GearFdbk,Driver.IgnFdbk
  Bus Selector2 : BusSelector  OutputSignals=Body.InertFrm.Cg.Disp.X,Body.InertFrm.Cg.Disp.Y,Body.InertFrm.Cg.Disp.Z,Body.InertFrm.Cg.Vel.Xdot,Body.InertFrm.Cg.Vel.Ydot,Body.InertFrm.Cg.Vel.Zdot,Body.InertFrm.Cg.Ang.phi,Body.InertFrm.Cg.Ang.theta,Body.InertFrm.Cg.Ang.psi,Body.InertFrm.Geom.Disp.X,Body.InertFrm.Geom.Disp.Y,Body.InertFrm.Geom.Disp.Z,Body.InertFrm.Geom.Vel.Xdot,Body.InertFrm.Geom.Vel.Ydot,Body.InertFrm.Geom.Vel.Zdot,Body.BdyFrm.Cg.Vel.xdot,Body.BdyFrm.Cg.Vel.ydot,Body.BdyFrm.Cg.Vel.zdot,Body.BdyFrm.Cg.AngVel.p,Body.BdyFrm.Cg.AngVel.q,Body.BdyFrm.Cg.AngVel.r,Body.BdyFrm.Cg.Acc.ax,Body.BdyFrm.Cg.Acc.ay,Body.BdyFrm.Cg.Acc.az,Body.BdyFrm.Cg.Acc.xddot,Body.BdyFrm.Cg.Acc.yddot,Body.BdyFrm.Cg.Acc.zddot,Body.BdyFrm.Cg.AngAcc.pdot,Body.BdyFrm.Cg.AngAcc.qdot,Body.BdyFrm.Cg.AngAcc.rdot
  Bus Selector3 : BusSelector  OutputSignals=Engine.EngSpdOut,Trans.Info.Trans.TransGear
  Constant : Constant  Value=0  OutDataTypeStr=Bus: VVCVehFdbkBUS  SampleTime=-1
  Data Type Conversion : DataTypeConversion  SaturateOnIntegerOverflow=off  RndMeth=Floor
  Data Type Conversion1 : DataTypeConversion  SaturateOnIntegerOverflow=off  RndMeth=Floor
  Data Type Conversion2 : DataTypeConversion  SaturateOnIntegerOverflow=off  RndMeth=Floor
  Rate Transition : RateTransition  Integrity=off
  Rate Transition1 : RateTransition  Integrity=off
  Rate Transition2 : RateTransition  Integrity=off
  Unit Conversion{1..8} (8 alike) : UnitConversion
  ExtVehFdbk : Outport
  wires:
  Constant/1 -> Bus Assignment/1
  Bus Assignment/1 -> ExtVehFdbk/1
  Bus Selector1/1 -> Unit Conversion2/1  "<SteerFdbk>"
  Bus Selector1/2 -> Bus Assignment/3  "<AccelFdbk>"
  Bus Selector1/3 -> Bus Assignment/4  "<DecelFdbk>"
  Bus Selector1/4 -> Data Type Conversion1/1  "<GearFdbk>"
  Bus Selector1/5 -> Data Type Conversion2/1  "<IgnFdbk>"
  Bus Selector3/1 -> Unit Conversion1/1  "<EngSpdOut>"
  Bus Selector3/2 -> Data Type Conversion/1  "<TransGear>"
  Data Type Conversion/1 -> Bus Assignment/8
  Data Type Conversion1/1 -> Bus Assignment/5
  Data Type Conversion2/1 -> Bus Assignment/6
  Unit Conversion1/1 -> Bus Assignment/7
  Unit Conversion2/1 -> Bus Assignment/2
  Bus Selector2/1 -> Bus Assignment/9  "<X>"
  Bus Selector2/2 -> Bus Assignment/10  "<Y>"
  Bus Selector2/3 -> Bus Assignment/11  "<Z>"
  Bus Selector2/4 -> Bus Assignment/12  "<Xdot>"
  Bus Selector2/5 -> Bus Assignment/13  "<Ydot>"
  Bus Selector2/6 -> Bus Assignment/14  "<Zdot>"
  Bus Selector2/7 -> Unit Conversion6/1  "<phi>"
  Bus Selector2/8 -> Unit Conversion7/1  "<theta>"
  Bus Selector2/9 -> Unit Conversion8/1  "<psi>"
  Bus Selector2/10 -> Bus Assignment/18  "<X>"
  Bus Selector2/11 -> Bus Assignment/19  "<Y>"
  Bus Selector2/12 -> Bus Assignment/20  "<Z>"
  Bus Selector2/13 -> Bus Assignment/21  "<Xdot>"
  Bus Selector2/14 -> Bus Assignment/22  "<Ydot>"
  Bus Selector2/15 -> Bus Assignment/23  "<Zdot>"
  Bus Selector2/16 -> Bus Assignment/24  "<xdot>"
  Bus Selector2/17 -> Bus Assignment/25  "<ydot>"
  Bus Selector2/18 -> Bus Assignment/26  "<zdot>"
  Bus Selector2/19 -> Bus Assignment/27  "<p>"
  Bus Selector2/20 -> Bus Assignment/28  "<q>"
  Bus Selector2/21 -> Bus Assignment/29  "<r>"
  Bus Selector2/22 -> Unit Conversion3/1  "<ax>"
  Bus Selector2/23 -> Unit Conversion4/1  "<ay>"
  Bus Selector2/24 -> Unit Conversion5/1  "<az>"
  Bus Selector2/25 -> Bus Assignment/33  "<xddot>"
  Bus Selector2/26 -> Bus Assignment/34  "<yddot>"
  Bus Selector2/27 -> Bus Assignment/35  "<zddot>"
  Bus Selector2/28 -> Bus Assignment/36  "<pdot>"
  Bus Selector2/29 -> Bus Assignment/37  "<qdot>"
  Bus Selector2/30 -> Bus Assignment/38  "<rdot>"
  Unit Conversion3/1 -> Bus Assignment/30
  Unit Conversion4/1 -> Bus Assignment/31
  Unit Conversion5/1 -> Bus Assignment/32
  Unit Conversion6/1 -> Bus Assignment/15
  Unit Conversion7/1 -> Bus Assignment/16
  Unit Conversion8/1 -> Bus Assignment/17
  VehFdbk/1 -> Rate Transition/1, Rate Transition2/1, Rate Transition1/1
  Rate Transition/1 -> Bus Selector1/1
  Rate Transition1/1 -> Bus Selector3/1
  Rate Transition2/1 -> Bus Selector2/1

== system ConfiguredHevMmVirtualVehicle/Visualization/ISO 15037-1:2006 ==
  VehFdbk : Inport
  Disabled : Subsystem  VariantControl=0
  Enabled : Subsystem  VariantControl=1

== system ConfiguredHevMmVirtualVehicle/Visualization/Performance Calculations ==
  VehSpd : Inport
  FuelVolFlow : Inport  Port=2
  BattPwr : Inport  Port=3
  Add : Sum
  Divide : Product  Inputs=*/
  Divide1 : Product  Inputs=*/
  Divide2 : Product  Inputs=*/
  Integrator : Integrator
  Integrator1 : Integrator
  L/100 Km Calc : Product  Inputs=/*
  Product : Product
  Rate Transition3 : RateTransition  Deterministic=off
  Saturation : Saturate  UpperLimit=Inf  LowerLimit=0.001  ZeroCross=off
  Saturation1 : Saturate  UpperLimit=Inf  LowerLimit=1e-3  ZeroCross=off
  Signal Specification5 : SignalSpecification  Unit=m/s
  Sqrt : Sqrt
  US EPA kwh/USgal equivalent : Constant  Value=33.7
  US MPG Calc : Product  Inputs=*/
  Unit Conversion5 : UnitConversion
  m to 100Km : Gain  Gain=1/1000/100
  m to mile : Gain  Gain=0.000621371
  m^3 per gal : Gain  Gain=0.00378541
  m^3 to L : Gain  Gain=1000
  m^3 to US Gal : Gain  Gain=264.172
  s per h : Constant  Value=3600
  w per kw : Constant  Value=1000
  US MPG : Outport  VectorParamsAs1DForOutWhenUnconnected=off
  L/100Km : Outport  Port=2  VectorParamsAs1DForOutWhenUnconnected=off
  wires:
  m^3 to US Gal/1 -> Saturation1/1
  m^3 to L/1 -> L/100 Km Calc/2
  Integrator/1 -> m to mile/1, m to 100Km/1
  m to mile/1 -> US MPG Calc/1
  FuelVolFlow/1 -> Add/1
  Integrator1/1 -> m^3 to US Gal/1, m^3 to L/1
  Saturation/1 -> L/100 Km Calc/1
  m to 100Km/1 -> Saturation/1
  L/100 Km Calc/1 -> L/100Km/1  "L/100Km"
  US MPG Calc/1 -> Rate Transition3/1
  Saturation1/1 -> US MPG Calc/2
  Rate Transition3/1 -> US MPG/1  "US MPG"
  w per kw/1 -> Divide/2
  Divide/1 -> Divide2/1
  Divide2/1 -> Divide1/1
  s per h/1 -> Divide1/2
  Divide1/1 -> m^3 per gal/1
  Add/1 -> Integrator1/1
  m^3 per gal/1 -> Add/2
  US EPA kwh/USgal equivalent/1 -> Divide2/2
  BattPwr/1 -> Divide/1
  Sqrt/1 -> Integrator/1
  Product/1 -> Sqrt/1
  Signal Specification5/1 -> Product/2, Product/1
  Unit Conversion5/1 -> Signal Specification5/1
  VehSpd/1 -> Unit Conversion5/1

== system ConfiguredHevMmVirtualVehicle/Visualization/Scope Type ==
  "VehFdbk " : Inport
  "Vis " : Inport  Port=2
  DLC : Subsystem  VariantControl=1
  None : Subsystem  VariantControl=0
  XYZ : Subsystem  VariantControl=2
  " Ref" : Outport  VectorParamsAs1DForOutWhenUnconnected=off

== system ConfiguredHevMmVirtualVehicle/Visualization/Vehicle XY Plotter ==
  "VehFdbk " : Inport
  "Ref " : Inport  Port=2
  Disabled : Subsystem  VariantControl=2
  XY View : Subsystem  VariantControl=0
  XY View Ref : Subsystem  VariantControl=1
  XY View Ref with One-Axle Trailer : Subsystem  VariantControl=3

== system ConfiguredHevMmVirtualVehicle/Driver Commands/Driver Commands/Dashboard Widgets ==
  note: Controls
  VehFdbk : Inport
  Hazards : LampBlock  LabelPosition=Hide  DefaultColor=[192.0, 192.0, 192.0]  Icon=Hazards
  High Beams : LampBlock  LabelPosition=Hide  DefaultColor=[192.0, 192.0, 192.0]  Icon=HighBeams
  Knob : KnobBlock  LabelPosition=Bottom  ScaleMin=-90  ScaleMax=90  TickInterval=30
  Low Beams : LampBlock  LabelPosition=Hide  DefaultColor=[192.0, 192.0, 192.0]  Icon=LowBeams
  Push Button : PushButtonBlock  ButtonText=Hazzard  ButtonType=Latch  Icon=Hazards  IconOnColor=[1.0, 0.0, 0.0]  IconOffColor=[0.50196078431372548, 0.50196078431372548, 0.50196078431372548]  IconColor=On  OffValue=0.000000
  Push Button1 : PushButtonBlock  ButtonText=Start / Stop  ButtonType=Latch  IconOnColor=[0.0, 1.0, 0.0]  IconOffColor=[0.0, 0.0, 0.0]  IconColor=On  OffValue=0.000000
  Rotary Switch : RotarySwitchBlock  LabelPosition=Bottom
  Rotary Switch1 : RotarySwitchBlock  LabelPosition=Bottom
  Rotary Switch2 : RotarySwitchBlock  LabelPosition=Bottom
  Slider : SliderBlock  LabelPosition=Bottom  ScaleMax=1  TickInterval=.2
  Slider1 : SliderBlock  LabelPosition=Bottom  ScaleMax=1  TickInterval=.2
  Turn Signal Left : LampBlock  LabelPosition=Hide  DefaultColor=[192.0, 192.0, 192.0]  Icon=TurnSignalLeft
  Turn Signal Right : LampBlock  LabelPosition=Hide  DefaultColor=[192.0, 192.0, 192.0]  Icon=TurnSignalRight
  Widget Sinks : Subsystem
  Widget Sources : Subsystem
  Driver : Outport  VectorParamsAs1DForOutWhenUnconnected=off
  wires:
  VehFdbk/1 -> Widget Sinks/1(VehFdbk)
  Widget Sources/1(Driver) -> Driver/1

== system ConfiguredHevMmVirtualVehicle/Driver Commands/Driver Commands/Game Wheel Hardware ==
  VehFdbk : Inport
  Add : Sum  Inputs=-+
  Bus Creator1 : BusCreator  Inputs=6
  Compare To Zero : simulink/Logic and Bit Operations/Compare To Zero  relop=~=  OutDataTypeStr=boolean
  Constant : Constant  Value=false
  Constant1 : Constant
  Constant2 : Constant
  Cont LPF : autolibutils/Cont LPF  wc=10*2*pi  AbsoluteTolerance=auto  aMode=6
  Cont LPF1 : autolibutils/Cont LPF  wc=10*2*pi  AbsoluteTolerance=auto  aMode=6
  Dead Zone : DeadZone  LowerValue=0  UpperValue=.01  ZeroCross=off
  Demux1 : Demux  Outputs=2
  Gain : Gain  Gain=.5
  Game Wheel Input Requires Simulink 3D Animation Signal dimensions and scaling are hardware dependent : sl3dlib/Simulation 3D/Hardware Interface/Simulation 3D Joystick  Commented=on  joyid=1  adjustports=off  forcefeed=off
  Manual Switch : ManualSwitch  CurrentSetting=0
  OR : Logic  Operator=OR  IconShape=distinctive  AllPortsSameDT=off  OutDataTypeStr=boolean
  Paddle Shift : Subsystem
  Selector : Selector  InputPortWidth=8  IndexOptions=Index vector (dialog)  Indices=[1]  OutputSizes=1
  Selector1 : Selector  InputPortWidth=8  IndexOptions=Index vector (dialog)  Indices=[2 3]  OutputSizes=1
  Signal Specification : SignalSpecification  Unit=1
  Signal Specification1 : SignalSpecification  Unit=1
  Signal Specification2 : SignalSpecification  Unit=1
  Signal Specification3 : SignalSpecification  Unit=rad
  Stick Shift : Subsystem
  Switch : Switch  Criteria=u2 ~= 0  SaturateOnIntegerOverflow=off  InputSameDT=off
  Terminator : Terminator
  To Virtual Bus : SignalConversion  ConversionOutput=Virtual bus  OverrideOpt=off
  Unit Delay : UnitDelay  SampleTime=-1  HasFrameUpgradeWarning=on
  VVCLightsCmd : Constant  Value=0  OutDataTypeStr=Bus: VVCLightsCmdBUS  SampleTime=-1
  Wheel Angle Limit [rad] : Gain  Gain=2*2*pi
  Driver : Outport  VectorParamsAs1DForOutWhenUnconnected=off
  wires:
  Stick Shift/1(Gear) -> Manual Switch/2
  Paddle Shift/1(Gear) -> Manual Switch/1
  Game Wheel Input Requires Simulink 3D Animation Signal dimensions and scaling are hardware dependent/2 -> Paddle Shift/1(Buttons), Stick Shift/1(Buttons)
  Game Wheel Input Requires Simulink 3D Animation Signal dimensions and scaling are hardware dependent/1 -> Selector/1, Selector1/1
  To Virtual Bus/1 -> Bus Creator1/6  "LightsCmd"
  VVCLightsCmd/1 -> To Virtual Bus/1
  Constant1/1 -> Add/2
  Cont LPF/1 -> Wheel Angle Limit [rad]/1
  Demux1/1 -> Signal Specification/1
  Cont LPF1/1 -> Dead Zone/1
  Manual Switch/1 -> Signal Specification2/1
  Wheel Angle Limit [rad]/1 -> Signal Specification3/1
  Demux1/2 -> Signal Specification1/1
  Add/1 -> Gain/1
  Selector/1 -> Cont LPF/1
  Dead Zone/1 -> Demux1/1
  Gain/1 -> Cont LPF1/1
  Constant/1 -> Bus Creator1/5  "IgnSwtch"
  Signal Specification1/1 -> Bus Creator1/3  "DecelCmd"
  Signal Specification/1 -> Bus Creator1/2  "AccelCmd"
  VehFdbk/1 -> Terminator/1
  Bus Creator1/1 -> Driver/1
  Signal Specification3/1 -> Bus Creator1/1  "SteerCmd"
  Signal Specification2/1 -> Bus Creator1/4  "GearCmd"
  OR/1 -> Unit Delay/1, Switch/2
  Selector1/1 -> Switch/1, Compare To Zero/1
  Compare To Zero/1 -> OR/1
  Unit Delay/1 -> OR/2
  Switch/1 -> Add/1
  Constant2/1 -> Switch/3
